simulink model "handwritten_sim"  (R2025b)
settings: Solver=ode23t  StartTime=0.0  StopTime=0.001  MaxStep=1e-06  RelTol=1e-3
libraries: fl_lib x9, nesl_utility x3
settings Model: Creator=devva  LastModifiedBy=devva
settings SimscapeCC: SimscapeLogType=all

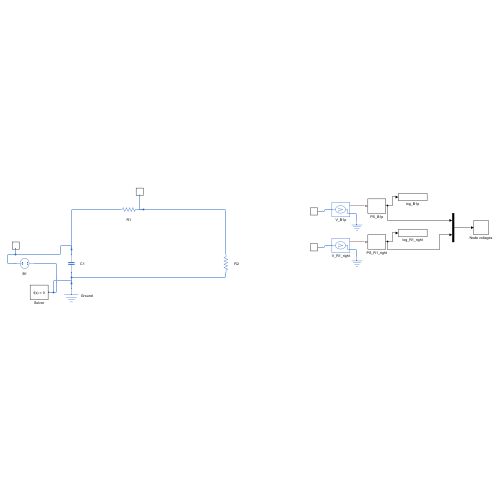
[thumbnail: Simulink's stored preview of the top-level diagram]
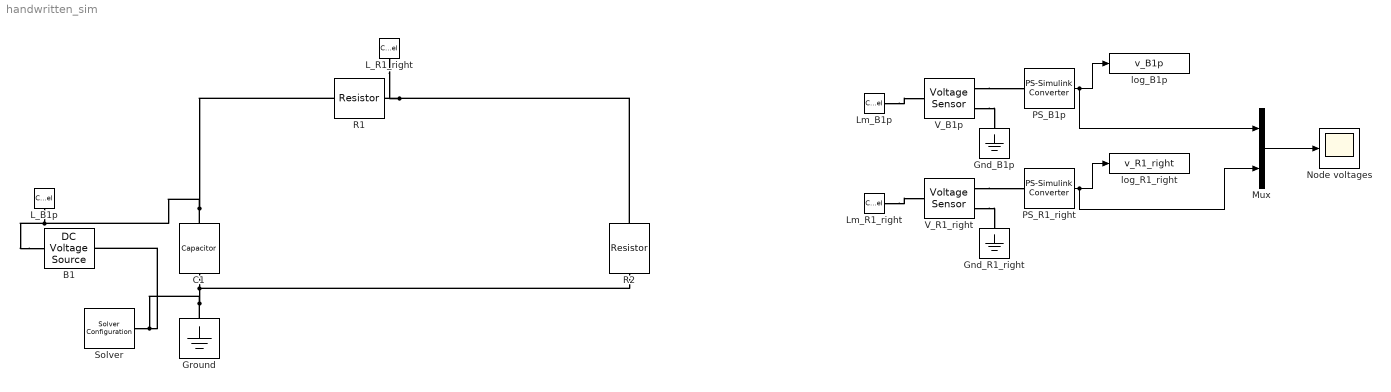
== system handwritten_sim ==
  B1 : fl_lib/Electrical/Electrical Sources/DC Voltage Source  v0=5 V
  C1 : fl_lib/Electrical/Electrical Elements/Capacitor  c=3e-06 F  r=1e-6 Ohm  g=0 1/Ohm  i_specify=off  i_priority=None  i=0 A  i_nominal_specify=off  i_nominal_value=1  i_nominal_unit=A  v_specify=off  v_priority=None  v=0 V  v_nominal_specify=off  v_nominal_value=1  v_nominal_unit=V  vc_specify=off  vc_priority=High  vc=0 V  vc_nominal_specify=off  vc_nominal_value=1  vc_nominal_unit=V
  Gnd_B1p : fl_lib/Electrical/Electrical Elements/Electrical Reference
  Gnd_R1_right : fl_lib/Electrical/Electrical Elements/Electrical Reference
  Ground : fl_lib/Electrical/Electrical Elements/Electrical Reference
  L_B1p : ConnectionLabel  Label=B1p
  L_R1_right : ConnectionLabel  Label=R1_right
  Lm_B1p : ConnectionLabel  Label=B1p
  Lm_R1_right : ConnectionLabel  Label=R1_right
  Mux : Mux  Inputs=2
  Node voltages : Scope
  PS_B1p : nesl_utility/PS-Simulink Converter  PhysicalDomain=network_engine_domain  SubClassName=ps_output  LeftPortType=input  RightPortType=output  PseudoPeriodic=off  Frequencies=[]  VectorFormat=inherit  Unit=inherit  AffineConversion=off
  PS_R1_right : nesl_utility/PS-Simulink Converter  PhysicalDomain=network_engine_domain  SubClassName=ps_output  LeftPortType=input  RightPortType=output  PseudoPeriodic=off  Frequencies=[]  VectorFormat=inherit  Unit=inherit  AffineConversion=off
  R1 : fl_lib/Electrical/Electrical Elements/Resistor  R=5 Ohm  i_specify=off  i_priority=None  i=0 A  i_nominal_specify=off  i_nominal_value=1  i_nominal_unit=A  v_specify=off  v_priority=None  v=0 V  v_nominal_specify=off  v_nominal_value=1  v_nominal_unit=V
  R2 : fl_lib/Electrical/Electrical Elements/Resistor  R=2 Ohm  i_specify=off  i_priority=None  i=0 A  i_nominal_specify=off  i_nominal_value=1  i_nominal_unit=A  v_specify=off  v_priority=None  v=0 V  v_nominal_specify=off  v_nominal_value=1  v_nominal_unit=V
  Solver : nesl_utility/Solver Configuration  PhysicalDomain=network_engine_domain  SubClassName=solver  LeftPortType=input  RightPortType=generic  Tones=[]  Harmonics=[]  SimulateNoise=off  Profile=off  UseLocalSampling=off  EnableSwitchedLinearOptims=on  FrequencyDomain=off  UseCCode=off  RelTol=0.001  AbsTol=0.001  MinStep=1e-09  ToWorkspace=off  RevertToSquareIcSolve=off  NumHomotopyIterations=100  PhasorMode=off  PhasorModeNumHarmonics=1  ConsistencySolver=NEWTON_XTOL_AFTER_FTOL  IndexReductionMethod=DerivativeReplacement  DoDC=off  ResidualTolerance=1e-09  ConsistencyTolSource=GLOBAL  ConsistencyAbsTol=0.001  ConsistencyRelTol=0.001  ConsistencyTolFactor=0.001  UseLocalSolver=off  LocalSolverChoice=NE_BACKWARD_EULER_ADVANCER  ResolveIndetEquations=on  FunctionEvalNumThread=1  LocalSolverSampleTime=0.001  DoFixedCost=off  MaxNonlinIter=3  MaxModeIter=2  ComputeImpulses=off  ImpulseIterations=2  LinearAlgebra=auto  LinearAlgebraNumThread=0  EquationFormulation=NE_TIME_EF  DelaysMemoryBudget=1024  AutomaticFiltering=on  FilteringTimeConstant=0.001  PartitionStorageMethod=AS_NEEDED  PartitionMemoryBudget=1024  PartitionMethod=ROBUST  MultibodyUseLocalSolver=off  MultibodyLocalSolverChoice=ODE1  MultibodyLocalSolverSampleTime=0.001
  V_B1p : fl_lib/Electrical/Electrical Sensors/Voltage Sensor
  V_R1_right : fl_lib/Electrical/Electrical Sensors/Voltage Sensor
  log_B1p : ToWorkspace  VariableName=v_B1p  SampleTime=-1
  log_R1_right : ToWorkspace  VariableName=v_R1_right  SampleTime=-1
  wires:
  PS_B1p/1 -> log_B1p/1, Mux/1
  PS_R1_right/1 -> log_R1_right/1, Mux/2
  Mux/1 -> Node voltages/1
  connections:
  V_B1p/RConn1 -- PS_B1p/LConn1
  Lm_B1p/LConn1 -- V_B1p/LConn1
  V_B1p/RConn2 -- Gnd_B1p/LConn1
  V_R1_right/RConn1 -- PS_R1_right/LConn1
  Lm_R1_right/LConn1 -- V_R1_right/LConn1
  V_R1_right/RConn2 -- Gnd_R1_right/LConn1
  B1/RConn1 -- Solver/RConn1 -- Ground/LConn1 -- C1/RConn1 -- R2/RConn1
  B1/LConn1 -- L_B1p/LConn1 -- C1/LConn1 -- R1/LConn1
  R1/RConn1 -- L_R1_right/LConn1 -- R2/LConn1
